simulink model "FlightComputer"  (R2024b)
settings: Solver=FixedStepDiscrete  StartTime=0.0  StopTime=10.0  FixedStep=0.01  RelTol=1e-3
settings Model: DataDictionary=FlightControl.sldd  EnableAccessToBaseWorkspace=off  Creator=enrico  LastModifiedBy=enrico
settings SolverCC: AutoInsertRateTranBlk=on
settings OptimizationCC: EnhancedBackFolding=on  PassReuseOutputArgsAs=Individual arguments  ZeroExternalMemoryAtStartup=off  ZeroInternalMemoryAtStartup=off  MaxStackSize=64  OptimizeBlockOrder=speed  DifferentSizesBufferReuse=on  OptimizationCustomize=off  EfficientTunableParamExpr=on
settings DebuggingCC: ParameterTunabilityLossMsg=error
settings HardwareCC: ProdBitPerPointer=32  ProdBitPerSizeT=32  ProdBitPerPtrDiffT=32  ProdLargestAtomicInteger=Long  ProdLargestAtomicFloat=Double  ProdWordSize=32  ProdHWDeviceType=ARM Compatible->ARM Cortex
settings SFSimCC: MATLABDynamicMemAlloc=off
settings RTWCC: Description=Embedded Coder  SystemTargetFile=ert.tlc  GenCodeOnly=on  TemplateMakefile=ert_default_tmf  Toolchain=Arduino ARM RP2040  BuildConfiguration=Faster Runs  DataTypeReplacement=CDataTypesFixedWidth
settings CodeAppCC: ForceParamTrailComments=on  IgnoreCustomStorageClasses=off  OperatorAnnotations=on  SimulinkDataObjDesc=on  SFDataObjDesc=on  InsertBlockDesc=on  StateflowObjectComments=on
settings ERTTargetCC: TargetLangStandard=C99 (ISO)  ExtMode=on  ExtModeTransport=3  ExtModeStaticAlloc=on  ExtModeStaticAllocSize=65536  ExtModeMexFile=ext_xcp  ExtModeIntrfLevel=Level2 - Open  InlinedParameterPlacement=Hierarchical  ERTCustomFileTemplate=example_file_process.tlc  IndentSize=4  MaxIdInt64=INT64_MAX  MinIdInt64=INT64_MIN  MaxIdUint64=UINT64_MAX  MaxIdInt32=INT32_MAX  MinIdInt32=INT32_MIN  MaxIdUint32=UINT32_MAX  MaxIdInt16=INT16_MAX  MinIdInt16=INT16_MIN  MaxIdUint16=UINT16_MAX  MaxIdInt8=INT8_MAX  MinIdInt8=INT8_MIN  MaxIdUint8=UINT8_MAX

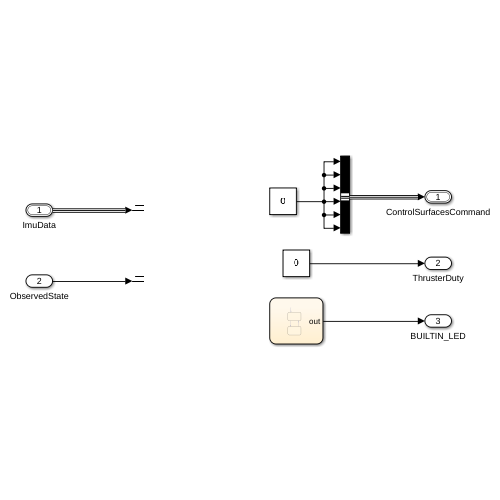
[thumbnail: Simulink's stored preview of the top-level diagram]
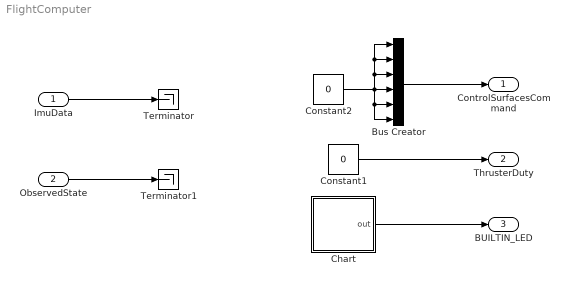
== system FlightComputer ==
  ImuData : Inport  OutDataTypeStr=Bus: ImuData
  ObservedState : Inport  Port=2
  Bus Creator : BusCreator  Inputs=6  OutDataTypeStr=Bus: ControlSurfaceData
      settings: InheritFromInputs=off
  Chart : Stateflow chart  TreatAsAtomicUnit=on
  Constant1 : Constant  Value=0
  Constant2 : Constant  Value=0  OutDataTypeStr=single
  Terminator : Terminator
  Terminator1 : Terminator
  ControlSurfacesCommand : Outport  OutDataTypeStr=Bus: ControlSurfaceData
  ThrusterDuty : Outport  Port=2  OutMin=0  OutMax=1  PortDimensions=1
  BUILTIN_LED : Outport  Port=3  OutMin=0  OutMax=1  PortDimensions=1
  wires:
  ImuData/1 -> Terminator/1
  ObservedState/1 -> Terminator1/1
  Bus Creator/1 -> ControlSurfacesCommand/1
  Constant1/1 -> ThrusterDuty/1
  Chart/1(out) -> BUILTIN_LED/1
  Constant2/1 -> Bus Creator/3, Bus Creator/1, Bus Creator/2, Bus Creator/4, Bus Creator/6, Bus Creator/5

== stateflow chart FlightComputer/Chart ==
  state OFF
    out = 0;
  state ON
    out = 1;
  (default) -> OFF
  OFF -> ON : [after(0.5, sec)]
  ON -> OFF : [after(0.5, sec)]
  data: out output
